simulink model "solar_battery_model"  (R2026a)
settings: Solver=VariableStepAuto  StopTime=30

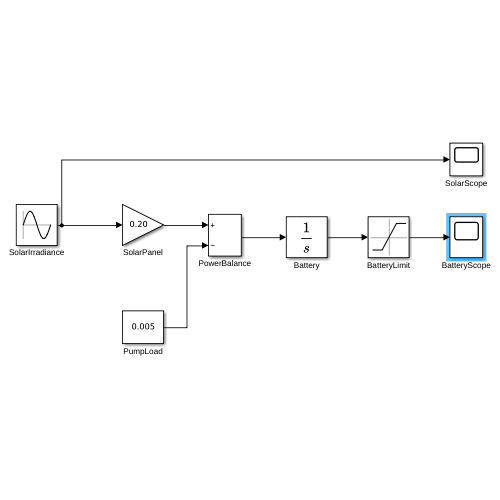
[thumbnail: Simulink's stored preview of the top-level diagram]
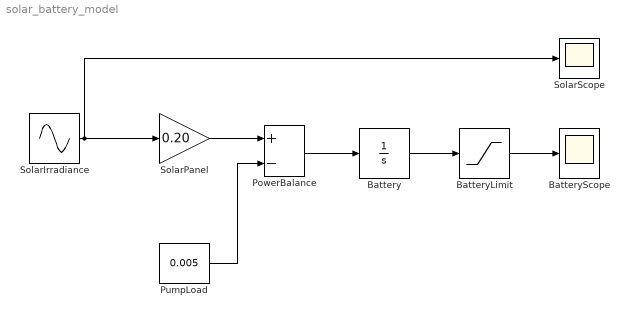
== system solar_battery_model ==
  Battery : Integrator  InitialCondition=12.4
  BatteryLimit : Saturate  UpperLimit=14.4  LowerLimit=10.5
  BatteryScope : Scope
      settings: ActiveDisplayYMinimum=12.150000000000002  ActiveDisplayYMaximum=14.65
  PowerBalance : Sum  Inputs=+-
  PumpLoad : Constant  Value=0.005
  SolarIrradiance : Sin  Amplitude=400  Bias=400  Frequency=0.2094  Phase=-1.5708  SampleTime=0
  SolarPanel : Gain  Gain=0.20
  SolarScope : Scope
      settings: ActiveDisplayYMinimum=-99.906786817579444  ActiveDisplayYMaximum=899.16108138520042
  wires:
  SolarIrradiance/1 -> SolarPanel/1, SolarScope/1
  SolarPanel/1 -> PowerBalance/1
  PumpLoad/1 -> PowerBalance/2
  PowerBalance/1 -> Battery/1
  Battery/1 -> BatteryLimit/1
  BatteryLimit/1 -> BatteryScope/1
